simulink model "ElectricalCoupling_testing"  (R2024b)
settings: Solver=FixedStepAuto  StartTime=0.0  StopTime=20  RelTol=1e-3
undefined symbols (not defined in the file): ac4b, c4e6, DiscIntNeverNeededParam
libraries: fl_lib x22, nesl_utility x21, ee_lib x5, simulink x3
(part 2 of 2)

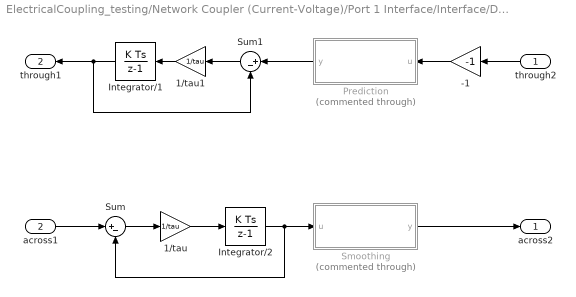
== system ElectricalCoupling_testing/Network Coupler (Current-Voltage)/Port 1 Interface/Interface/Discrete ==
  through2 : Inport
  across1 : Inport  Port=2
  -1 : Gain  Gain=-1  SaturateOnIntegerOverflow=on  OutDataTypeStr=Inherit: Same as input  ParamDataTypeStr=Inherit: Same as input
  1/tau : Gain  Gain=1/tau  SaturateOnIntegerOverflow=on  OutDataTypeStr=Inherit: Same as input  ParamDataTypeStr=Inherit: Same as input
  1/tau1 : Gain  Gain=1/tau  SaturateOnIntegerOverflow=on  OutDataTypeStr=Inherit: Same as input  ParamDataTypeStr=Inherit: Same as input
  Integrator/1 : DiscreteIntegrator  InitialCondition=i0  SampleTime=h1  ICPrevOutput=DiscIntNeverNeededParam  ICPrevScaledInput=DiscIntNeverNeededParam
  Integrator/2 : DiscreteIntegrator  InitialCondition=v0  SampleTime=h1  ICPrevOutput=DiscIntNeverNeededParam  ICPrevScaledInput=DiscIntNeverNeededParam
  Prediction : Subsystem  Commented=through  mask(Prediction (slow->fast)){h2=h2, h1=h1}
      mask prompts: h2 "physmod:simscape:couplers:SimscapeNetworkCouplersLib:PortUDiscreteSampleTimes_MP"; h1 "physmod:simscape:couplers:SimscapeNetworkCouplersLib:PortYDiscreteSampleTimes_MP"
      mask help: physmod:simscape:couplers:SimscapeNetworkCouplersLib:Predictionslowfast_MD
      mask DialogControl h2 Prompt: Port u discrete sample time (s)
      mask DialogControl h1 Prompt: Port y discrete sample time (s)
  Smoothing : Subsystem  Commented=through  mask(Smoothing (fast->slow)){nSmooth=nSmooth, h1=h1, smoothing0=v0}
      mask prompts: nSmooth "physmod:simscape:couplers:SimscapeNetworkCouplersLib:NumberOfSamplesOverWhichToSmooth_MP"; h1 "physmod:simscape:couplers:SimscapeNetworkCouplersLib:PortUDiscreteSampleTimes_MP"; smoothing0 "physmod:simscape:couplers:SimscapeNetworkCouplersLib:InitialOutput_MP"
      mask help: physmod:simscape:couplers:SimscapeNetworkCouplersLib:Smoothingfastslow_MD
      mask DialogControl nSmooth Prompt: Number of samples over which to smooth
      mask DialogControl h1 Prompt: Port u discrete sample time (s)
      mask DialogControl smoothing0 Prompt: Initial output
  Sum : Sum  Inputs=|+-  InputSameDT=on  SaturateOnIntegerOverflow=on  OutDataTypeStr=Inherit: Same as first input
  Sum1 : Sum  Inputs=|+-  InputSameDT=on  SaturateOnIntegerOverflow=on  OutDataTypeStr=Inherit: Same as first input
  across2 : Outport
  through1 : Outport  Port=2
  wires:
  Smoothing/1(y) -> across2/1
  -1/1 -> Prediction/1(u)
  through2/1 -> -1/1
  Prediction/1(y) -> Sum1/1
  Sum1/1 -> 1/tau1/1
  Integrator/1/1 -> through1/1, Sum1/2
  Integrator/2/1 -> Sum/2, Smoothing/1(u)
  Sum/1 -> 1/tau/1
  1/tau1/1 -> Integrator/1/1
  1/tau/1 -> Integrator/2/1
  across1/1 -> Sum/1

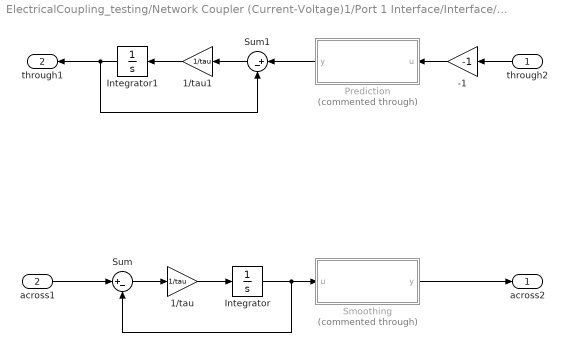
== system ElectricalCoupling_testing/Network Coupler (Current-Voltage)1/Port 1 Interface/Interface/Continuous ==
  through2 : Inport
  across1 : Inport  Port=2
  -1 : Gain  Gain=-1  SaturateOnIntegerOverflow=on  OutDataTypeStr=Inherit: Same as input  ParamDataTypeStr=Inherit: Same as input
  1/tau : Gain  Gain=1/tau  SaturateOnIntegerOverflow=on  OutDataTypeStr=Inherit: Same as input  ParamDataTypeStr=Inherit: Same as input
  1/tau1 : Gain  Gain=1/tau  SaturateOnIntegerOverflow=on  OutDataTypeStr=Inherit: Same as input  ParamDataTypeStr=Inherit: Same as input
  Integrator : Integrator  InitialCondition=v0
  Integrator1 : Integrator  InitialCondition=i0
  Prediction : Subsystem  Commented=through  mask(Prediction (discrete->continuous)){h2=h2}
      mask prompts: h2 "physmod:simscape:couplers:SimscapeNetworkCouplersLib:PortUDiscreteSampleTimes_MP"
      mask help: physmod:simscape:couplers:SimscapeNetworkCouplersLib:Predictiondiscretecontinuous_MD
      mask DialogControl h2 Prompt: Port u discrete sample time (s)
  Smoothing : Subsystem  Commented=through  mask(Smoothing (continuous->discrete)){tsSmoothing=tsSmoothing, smoothing0=v0}
      mask prompts: tsSmoothing "physmod:simscape:couplers:SimscapeNetworkCouplersLib:SmoothingTimeConstants_MP"; smoothing0 "physmod:simscape:couplers:SimscapeNetworkCouplersLib:InitialOutput_MP"
      mask help: physmod:simscape:couplers:SimscapeNetworkCouplersLib:Smoothingcontinuousdiscrete_MD
      mask DialogControl tsSmoothing Prompt: Smoothing time constant (s)
      mask DialogControl smoothing0 Prompt: Initial output
  Sum : Sum  Inputs=|+-  InputSameDT=on  SaturateOnIntegerOverflow=on  OutDataTypeStr=Inherit: Same as first input
  Sum1 : Sum  Inputs=|+-  InputSameDT=on  SaturateOnIntegerOverflow=on  OutDataTypeStr=Inherit: Same as first input
  across2 : Outport
  through1 : Outport  Port=2
  wires:
  Prediction/1(y) -> Sum1/1
  Sum1/1 -> 1/tau1/1
  1/tau1/1 -> Integrator1/1
  Integrator1/1 -> through1/1, Sum1/2
  across1/1 -> Sum/1
  Integrator/1 -> Smoothing/1(u), Sum/2
  Sum/1 -> 1/tau/1
  1/tau/1 -> Integrator/1
  through2/1 -> -1/1
  -1/1 -> Prediction/1(u)
  Smoothing/1(y) -> across2/1

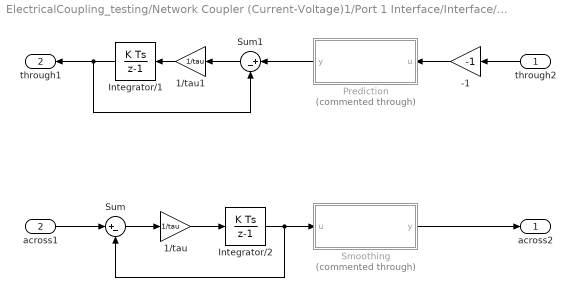
== system ElectricalCoupling_testing/Network Coupler (Current-Voltage)1/Port 1 Interface/Interface/Discrete ==
  through2 : Inport
  across1 : Inport  Port=2
  -1 : Gain  Gain=-1  SaturateOnIntegerOverflow=on  OutDataTypeStr=Inherit: Same as input  ParamDataTypeStr=Inherit: Same as input
  1/tau : Gain  Gain=1/tau  SaturateOnIntegerOverflow=on  OutDataTypeStr=Inherit: Same as input  ParamDataTypeStr=Inherit: Same as input
  1/tau1 : Gain  Gain=1/tau  SaturateOnIntegerOverflow=on  OutDataTypeStr=Inherit: Same as input  ParamDataTypeStr=Inherit: Same as input
  Integrator/1 : DiscreteIntegrator  InitialCondition=i0  SampleTime=h1  ICPrevOutput=DiscIntNeverNeededParam  ICPrevScaledInput=DiscIntNeverNeededParam
  Integrator/2 : DiscreteIntegrator  InitialCondition=v0  SampleTime=h1  ICPrevOutput=DiscIntNeverNeededParam  ICPrevScaledInput=DiscIntNeverNeededParam
  Prediction : Subsystem  Commented=through  mask(Prediction (slow->fast)){h2=h2, h1=h1}
      mask prompts: h2 "physmod:simscape:couplers:SimscapeNetworkCouplersLib:PortUDiscreteSampleTimes_MP"; h1 "physmod:simscape:couplers:SimscapeNetworkCouplersLib:PortYDiscreteSampleTimes_MP"
      mask help: physmod:simscape:couplers:SimscapeNetworkCouplersLib:Predictionslowfast_MD
      mask DialogControl h2 Prompt: Port u discrete sample time (s)
      mask DialogControl h1 Prompt: Port y discrete sample time (s)
  Smoothing : Subsystem  Commented=through  mask(Smoothing (fast->slow)){nSmooth=nSmooth, h1=h1, smoothing0=v0}
      mask prompts: nSmooth "physmod:simscape:couplers:SimscapeNetworkCouplersLib:NumberOfSamplesOverWhichToSmooth_MP"; h1 "physmod:simscape:couplers:SimscapeNetworkCouplersLib:PortUDiscreteSampleTimes_MP"; smoothing0 "physmod:simscape:couplers:SimscapeNetworkCouplersLib:InitialOutput_MP"
      mask help: physmod:simscape:couplers:SimscapeNetworkCouplersLib:Smoothingfastslow_MD
      mask DialogControl nSmooth Prompt: Number of samples over which to smooth
      mask DialogControl h1 Prompt: Port u discrete sample time (s)
      mask DialogControl smoothing0 Prompt: Initial output
  Sum : Sum  Inputs=|+-  InputSameDT=on  SaturateOnIntegerOverflow=on  OutDataTypeStr=Inherit: Same as first input
  Sum1 : Sum  Inputs=|+-  InputSameDT=on  SaturateOnIntegerOverflow=on  OutDataTypeStr=Inherit: Same as first input
  across2 : Outport
  through1 : Outport  Port=2
  wires:
  across1/1 -> Sum/1
  1/tau/1 -> Integrator/2/1
  1/tau1/1 -> Integrator/1/1
  Sum/1 -> 1/tau/1
  Integrator/2/1 -> Smoothing/1(u), Sum/2
  Integrator/1/1 -> Sum1/2, through1/1
  Sum1/1 -> 1/tau1/1
  Prediction/1(y) -> Sum1/1
  through2/1 -> -1/1
  -1/1 -> Prediction/1(u)
  Smoothing/1(y) -> across2/1

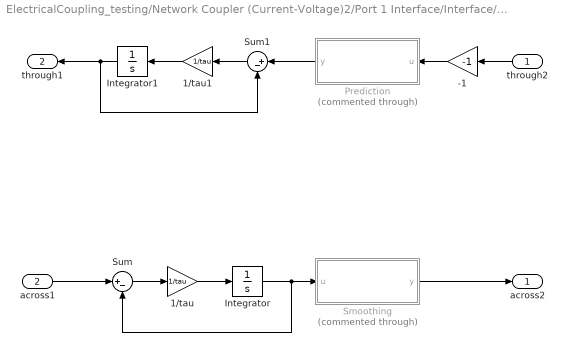
== system ElectricalCoupling_testing/Network Coupler (Current-Voltage)2/Port 1 Interface/Interface/Continuous ==
  through2 : Inport
  across1 : Inport  Port=2
  -1 : Gain  Gain=-1  SaturateOnIntegerOverflow=on  OutDataTypeStr=Inherit: Same as input  ParamDataTypeStr=Inherit: Same as input
  1/tau : Gain  Gain=1/tau  SaturateOnIntegerOverflow=on  OutDataTypeStr=Inherit: Same as input  ParamDataTypeStr=Inherit: Same as input
  1/tau1 : Gain  Gain=1/tau  SaturateOnIntegerOverflow=on  OutDataTypeStr=Inherit: Same as input  ParamDataTypeStr=Inherit: Same as input
  Integrator : Integrator  InitialCondition=v0
  Integrator1 : Integrator  InitialCondition=i0
  Prediction : Subsystem  Commented=through  mask(Prediction (discrete->continuous)){h2=h2}
      mask prompts: h2 "physmod:simscape:couplers:SimscapeNetworkCouplersLib:PortUDiscreteSampleTimes_MP"
      mask help: physmod:simscape:couplers:SimscapeNetworkCouplersLib:Predictiondiscretecontinuous_MD
      mask DialogControl h2 Prompt: Port u discrete sample time (s)
  Smoothing : Subsystem  Commented=through  mask(Smoothing (continuous->discrete)){tsSmoothing=tsSmoothing, smoothing0=v0}
      mask prompts: tsSmoothing "physmod:simscape:couplers:SimscapeNetworkCouplersLib:SmoothingTimeConstants_MP"; smoothing0 "physmod:simscape:couplers:SimscapeNetworkCouplersLib:InitialOutput_MP"
      mask help: physmod:simscape:couplers:SimscapeNetworkCouplersLib:Smoothingcontinuousdiscrete_MD
      mask DialogControl tsSmoothing Prompt: Smoothing time constant (s)
      mask DialogControl smoothing0 Prompt: Initial output
  Sum : Sum  Inputs=|+-  InputSameDT=on  SaturateOnIntegerOverflow=on  OutDataTypeStr=Inherit: Same as first input
  Sum1 : Sum  Inputs=|+-  InputSameDT=on  SaturateOnIntegerOverflow=on  OutDataTypeStr=Inherit: Same as first input
  across2 : Outport
  through1 : Outport  Port=2
  wires:
  Smoothing/1(y) -> across2/1
  -1/1 -> Prediction/1(u)
  through2/1 -> -1/1
  1/tau/1 -> Integrator/1
  Sum/1 -> 1/tau/1
  Integrator/1 -> Sum/2, Smoothing/1(u)
  across1/1 -> Sum/1
  Integrator1/1 -> Sum1/2, through1/1
  1/tau1/1 -> Integrator1/1
  Sum1/1 -> 1/tau1/1
  Prediction/1(y) -> Sum1/1

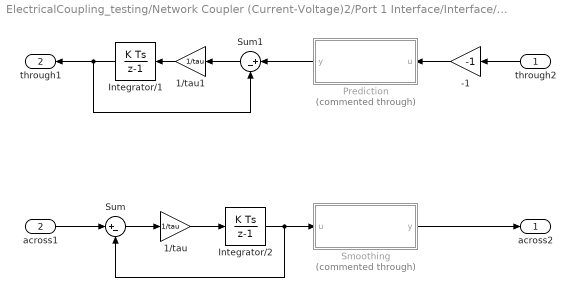
== system ElectricalCoupling_testing/Network Coupler (Current-Voltage)2/Port 1 Interface/Interface/Discrete ==
  through2 : Inport
  across1 : Inport  Port=2
  -1 : Gain  Gain=-1  SaturateOnIntegerOverflow=on  OutDataTypeStr=Inherit: Same as input  ParamDataTypeStr=Inherit: Same as input
  1/tau : Gain  Gain=1/tau  SaturateOnIntegerOverflow=on  OutDataTypeStr=Inherit: Same as input  ParamDataTypeStr=Inherit: Same as input
  1/tau1 : Gain  Gain=1/tau  SaturateOnIntegerOverflow=on  OutDataTypeStr=Inherit: Same as input  ParamDataTypeStr=Inherit: Same as input
  Integrator/1 : DiscreteIntegrator  InitialCondition=i0  SampleTime=h1  ICPrevOutput=DiscIntNeverNeededParam  ICPrevScaledInput=DiscIntNeverNeededParam
  Integrator/2 : DiscreteIntegrator  InitialCondition=v0  SampleTime=h1  ICPrevOutput=DiscIntNeverNeededParam  ICPrevScaledInput=DiscIntNeverNeededParam
  Prediction : Subsystem  Commented=through  mask(Prediction (slow->fast)){h2=h2, h1=h1}
      mask prompts: h2 "physmod:simscape:couplers:SimscapeNetworkCouplersLib:PortUDiscreteSampleTimes_MP"; h1 "physmod:simscape:couplers:SimscapeNetworkCouplersLib:PortYDiscreteSampleTimes_MP"
      mask help: physmod:simscape:couplers:SimscapeNetworkCouplersLib:Predictionslowfast_MD
      mask DialogControl h2 Prompt: Port u discrete sample time (s)
      mask DialogControl h1 Prompt: Port y discrete sample time (s)
  Smoothing : Subsystem  Commented=through  mask(Smoothing (fast->slow)){nSmooth=nSmooth, h1=h1, smoothing0=v0}
      mask prompts: nSmooth "physmod:simscape:couplers:SimscapeNetworkCouplersLib:NumberOfSamplesOverWhichToSmooth_MP"; h1 "physmod:simscape:couplers:SimscapeNetworkCouplersLib:PortUDiscreteSampleTimes_MP"; smoothing0 "physmod:simscape:couplers:SimscapeNetworkCouplersLib:InitialOutput_MP"
      mask help: physmod:simscape:couplers:SimscapeNetworkCouplersLib:Smoothingfastslow_MD
      mask DialogControl nSmooth Prompt: Number of samples over which to smooth
      mask DialogControl h1 Prompt: Port u discrete sample time (s)
      mask DialogControl smoothing0 Prompt: Initial output
  Sum : Sum  Inputs=|+-  InputSameDT=on  SaturateOnIntegerOverflow=on  OutDataTypeStr=Inherit: Same as first input
  Sum1 : Sum  Inputs=|+-  InputSameDT=on  SaturateOnIntegerOverflow=on  OutDataTypeStr=Inherit: Same as first input
  across2 : Outport
  through1 : Outport  Port=2
  wires:
  Smoothing/1(y) -> across2/1
  -1/1 -> Prediction/1(u)
  through2/1 -> -1/1
  Prediction/1(y) -> Sum1/1
  Sum1/1 -> 1/tau1/1
  Integrator/1/1 -> through1/1, Sum1/2
  Integrator/2/1 -> Sum/2, Smoothing/1(u)
  Sum/1 -> 1/tau/1
  1/tau1/1 -> Integrator/1/1
  1/tau/1 -> Integrator/2/1
  across1/1 -> Sum/1

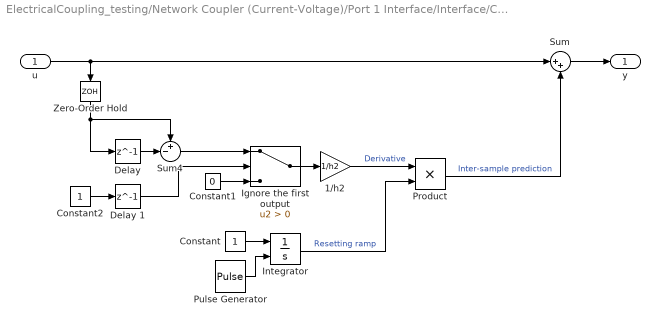
== system ElectricalCoupling_testing/Network Coupler (Current-Voltage)/Port 1 Interface/Interface/Continuous/Prediction ==
  u : Inport
  1/h2 : Gain  Gain=1/h2
  Constant : Constant  SampleTime=h2
  Constant1 : Constant  Value=0  SampleTime=h2
  Constant2 : Constant  SampleTime=h2
  "Delay " : Delay  DelayLength=1  SampleTime=h2
  Delay 1 : Delay  DelayLength=1  SampleTime=h2
  Ignore the first output : Switch  Criteria=u2 > Threshold  SaturateOnIntegerOverflow=off  InputSameDT=off
  Integrator : Integrator  ExternalReset=either  LimitOutput=on  UpperSaturationLimit=1  LowerSaturationLimit=0
  Product : Product
  Pulse Generator : DiscretePulseGenerator  SampleTime=h2
  Sum : Sum  Inputs=|++
  Sum4 : Sum  Inputs=+-|
  Zero-Order Hold : ZeroOrderHold  SampleTime=h2
  y : Outport
  wires:
  Constant2/1 -> Delay 1/1
  Delay 1/1 -> Ignore the first output/2
  Constant1/1 -> Ignore the first output/3
  Sum4/1 -> Ignore the first output/1
  Ignore the first output/1 -> 1/h2/1
  Pulse Generator/1 -> Integrator/2
  Constant/1 -> Integrator/1
  Integrator/1 -> Product/2  "Resetting ramp"
  Sum/1 -> y/1
  1/h2/1 -> Product/1  "Derivative"
  "Delay "/1 -> Sum4/2
  u/1 -> Zero-Order Hold/1, Sum/1
  Zero-Order Hold/1 -> "Delay "/1, Sum4/1
  Product/1 -> Sum/2  "Inter-sample prediction"

== system ElectricalCoupling_testing/Network Coupler (Current-Voltage)/Port 1 Interface/Interface/Continuous/Smoothing ==
  u : Inport
  Gain : Gain  Gain=1/tsSmoothing
  Integrator : Integrator  InitialCondition=smoothing0
  Sum : Sum  Inputs=|+-
  y : Outport
  wires:
  Sum/1 -> Gain/1
  Gain/1 -> Integrator/1
  Integrator/1 -> y/1, Sum/2
  u/1 -> Sum/1

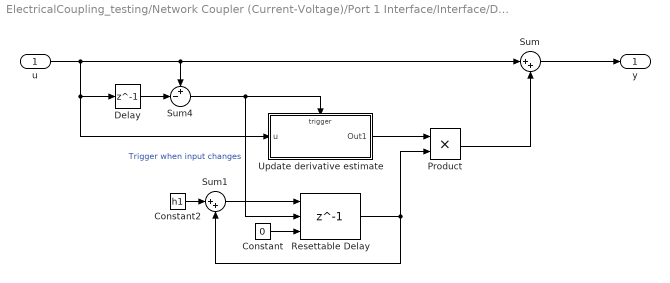
== system ElectricalCoupling_testing/Network Coupler (Current-Voltage)/Port 1 Interface/Interface/Discrete/Prediction ==
  u : Inport
  Constant : Constant  Value=0  SampleTime=h1
  Constant2 : Constant  Value=h1  SampleTime=h1
  "Delay " : Delay  DelayLength=1  SampleTime=h1
  Product : Product
  Resettable Delay : Delay  DelayLength=1  InitialConditionSource=Input port  ExternalReset=Rising  SampleTime=h1
      settings: InputPortMap=u0,r5,p4
  Sum : Sum  Inputs=|++
  Sum1 : Sum  Inputs=|++
  Sum4 : Sum  Inputs=+-|
  Update derivative estimate : Subsystem  TreatAsAtomicUnit=on
  y : Outport
  wires:
  Update derivative estimate/1(Out1) -> Product/1
  u/1 -> Sum/1, Sum4/1, Update derivative estimate/1(u), "Delay "/1
  "Delay "/1 -> Sum4/2
  Sum4/1 -> Update derivative estimate/Trigger, Resettable Delay/2  "Trigger when input changes"
  Sum1/1 -> Resettable Delay/1
  Resettable Delay/1 -> Product/2, Sum1/2
  Constant2/1 -> Sum1/1
  Constant/1 -> Resettable Delay/3
  Sum/1 -> y/1
  Product/1 -> Sum/2

== system ElectricalCoupling_testing/Network Coupler (Current-Voltage)/Port 1 Interface/Interface/Discrete/Smoothing ==
  u : Inport
  Gain : Gain  Gain=1/nSmooth
  Sum of Elements : Sum  Inputs=+
  Tapped Delay : simulink/Discrete/Tapped Delay  vinit=smoothing0  samptime=h1  NumDelays=nSmooth  DelayOrder=Oldest  includeCurrent=off
  y : Outport
  wires:
  u/1 -> Tapped Delay/1
  Tapped Delay/1 -> Sum of Elements/1
  Sum of Elements/1 -> Gain/1
  Gain/1 -> y/1

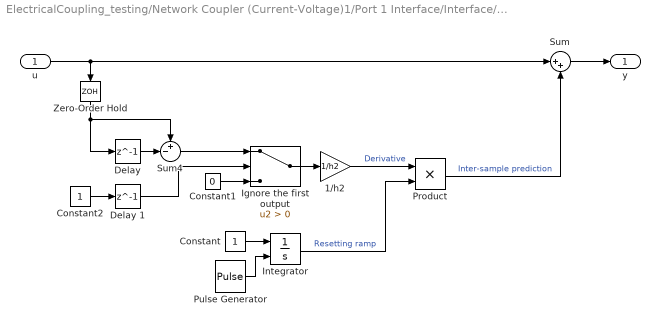
== system ElectricalCoupling_testing/Network Coupler (Current-Voltage)1/Port 1 Interface/Interface/Continuous/Prediction ==
  u : Inport
  1/h2 : Gain  Gain=1/h2
  Constant : Constant  SampleTime=h2
  Constant1 : Constant  Value=0  SampleTime=h2
  Constant2 : Constant  SampleTime=h2
  "Delay " : Delay  DelayLength=1  SampleTime=h2
  Delay 1 : Delay  DelayLength=1  SampleTime=h2
  Ignore the first output : Switch  Criteria=u2 > Threshold  SaturateOnIntegerOverflow=off  InputSameDT=off
  Integrator : Integrator  ExternalReset=either  LimitOutput=on  UpperSaturationLimit=1  LowerSaturationLimit=0
  Product : Product
  Pulse Generator : DiscretePulseGenerator  SampleTime=h2
  Sum : Sum  Inputs=|++
  Sum4 : Sum  Inputs=+-|
  Zero-Order Hold : ZeroOrderHold  SampleTime=h2
  y : Outport
  wires:
  Product/1 -> Sum/2  "Inter-sample prediction"
  Zero-Order Hold/1 -> Sum4/1, "Delay "/1
  u/1 -> Sum/1, Zero-Order Hold/1
  "Delay "/1 -> Sum4/2
  1/h2/1 -> Product/1  "Derivative"
  Sum/1 -> y/1
  Integrator/1 -> Product/2  "Resetting ramp"
  Constant/1 -> Integrator/1
  Pulse Generator/1 -> Integrator/2
  Ignore the first output/1 -> 1/h2/1
  Sum4/1 -> Ignore the first output/1
  Constant1/1 -> Ignore the first output/3
  Delay 1/1 -> Ignore the first output/2
  Constant2/1 -> Delay 1/1

== system ElectricalCoupling_testing/Network Coupler (Current-Voltage)1/Port 1 Interface/Interface/Continuous/Smoothing ==
  u : Inport
  Gain : Gain  Gain=1/tsSmoothing
  Integrator : Integrator  InitialCondition=smoothing0
  Sum : Sum  Inputs=|+-
  y : Outport
  wires:
  u/1 -> Sum/1
  Integrator/1 -> Sum/2, y/1
  Gain/1 -> Integrator/1
  Sum/1 -> Gain/1

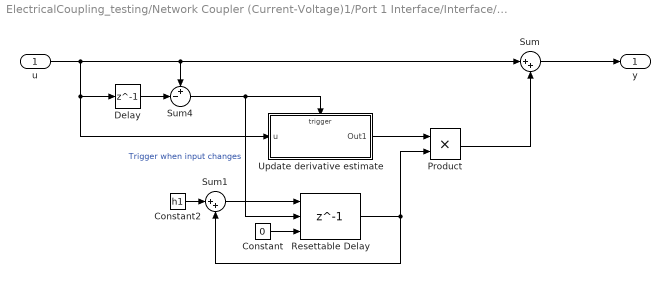
== system ElectricalCoupling_testing/Network Coupler (Current-Voltage)1/Port 1 Interface/Interface/Discrete/Prediction ==
  u : Inport
  Constant : Constant  Value=0  SampleTime=h1
  Constant2 : Constant  Value=h1  SampleTime=h1
  "Delay " : Delay  DelayLength=1  SampleTime=h1
  Product : Product
  Resettable Delay : Delay  DelayLength=1  InitialConditionSource=Input port  ExternalReset=Rising  SampleTime=h1
      settings: InputPortMap=u0,r5,p4
  Sum : Sum  Inputs=|++
  Sum1 : Sum  Inputs=|++
  Sum4 : Sum  Inputs=+-|
  Update derivative estimate : Subsystem  TreatAsAtomicUnit=on
  y : Outport
  wires:
  Product/1 -> Sum/2
  Sum/1 -> y/1
  Constant/1 -> Resettable Delay/3
  Constant2/1 -> Sum1/1
  Resettable Delay/1 -> Sum1/2, Product/2
  Sum1/1 -> Resettable Delay/1
  Sum4/1 -> Resettable Delay/2, Update derivative estimate/Trigger  "Trigger when input changes"
  "Delay "/1 -> Sum4/2
  u/1 -> "Delay "/1, Update derivative estimate/1(u), Sum4/1, Sum/1
  Update derivative estimate/1(Out1) -> Product/1

== system ElectricalCoupling_testing/Network Coupler (Current-Voltage)1/Port 1 Interface/Interface/Discrete/Smoothing ==
  u : Inport
  Gain : Gain  Gain=1/nSmooth
  Sum of Elements : Sum  Inputs=+
  Tapped Delay : simulink/Discrete/Tapped Delay  vinit=smoothing0  samptime=h1  NumDelays=nSmooth  DelayOrder=Oldest  includeCurrent=off
  y : Outport
  wires:
  Gain/1 -> y/1
  Sum of Elements/1 -> Gain/1
  Tapped Delay/1 -> Sum of Elements/1
  u/1 -> Tapped Delay/1

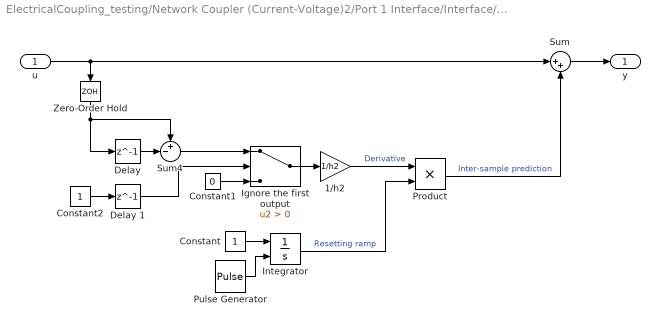
== system ElectricalCoupling_testing/Network Coupler (Current-Voltage)2/Port 1 Interface/Interface/Continuous/Prediction ==
  u : Inport
  1/h2 : Gain  Gain=1/h2
  Constant : Constant  SampleTime=h2
  Constant1 : Constant  Value=0  SampleTime=h2
  Constant2 : Constant  SampleTime=h2
  "Delay " : Delay  DelayLength=1  SampleTime=h2
  Delay 1 : Delay  DelayLength=1  SampleTime=h2
  Ignore the first output : Switch  Criteria=u2 > Threshold  SaturateOnIntegerOverflow=off  InputSameDT=off
  Integrator : Integrator  ExternalReset=either  LimitOutput=on  UpperSaturationLimit=1  LowerSaturationLimit=0
  Product : Product
  Pulse Generator : DiscretePulseGenerator  SampleTime=h2
  Sum : Sum  Inputs=|++
  Sum4 : Sum  Inputs=+-|
  Zero-Order Hold : ZeroOrderHold  SampleTime=h2
  y : Outport
  wires:
  Constant2/1 -> Delay 1/1
  Delay 1/1 -> Ignore the first output/2
  Constant1/1 -> Ignore the first output/3
  Sum4/1 -> Ignore the first output/1
  Ignore the first output/1 -> 1/h2/1
  Pulse Generator/1 -> Integrator/2
  Constant/1 -> Integrator/1
  Integrator/1 -> Product/2  "Resetting ramp"
  Sum/1 -> y/1
  1/h2/1 -> Product/1  "Derivative"
  "Delay "/1 -> Sum4/2
  u/1 -> Zero-Order Hold/1, Sum/1
  Zero-Order Hold/1 -> "Delay "/1, Sum4/1
  Product/1 -> Sum/2  "Inter-sample prediction"

== system ElectricalCoupling_testing/Network Coupler (Current-Voltage)2/Port 1 Interface/Interface/Continuous/Smoothing ==
  u : Inport
  Gain : Gain  Gain=1/tsSmoothing
  Integrator : Integrator  InitialCondition=smoothing0
  Sum : Sum  Inputs=|+-
  y : Outport
  wires:
  Sum/1 -> Gain/1
  Gain/1 -> Integrator/1
  Integrator/1 -> y/1, Sum/2
  u/1 -> Sum/1

== system ElectricalCoupling_testing/Network Coupler (Current-Voltage)2/Port 1 Interface/Interface/Discrete/Prediction ==
  u : Inport
  Constant : Constant  Value=0  SampleTime=h1
  Constant2 : Constant  Value=h1  SampleTime=h1
  "Delay " : Delay  DelayLength=1  SampleTime=h1
  Product : Product
  Resettable Delay : Delay  DelayLength=1  InitialConditionSource=Input port  ExternalReset=Rising  SampleTime=h1
      settings: InputPortMap=u0,r5,p4
  Sum : Sum  Inputs=|++
  Sum1 : Sum  Inputs=|++
  Sum4 : Sum  Inputs=+-|
  Update derivative estimate : Subsystem  TreatAsAtomicUnit=on
  y : Outport
  wires:
  Update derivative estimate/1(Out1) -> Product/1
  u/1 -> Sum/1, Sum4/1, Update derivative estimate/1(u), "Delay "/1
  "Delay "/1 -> Sum4/2
  Sum4/1 -> Update derivative estimate/Trigger, Resettable Delay/2  "Trigger when input changes"
  Sum1/1 -> Resettable Delay/1
  Resettable Delay/1 -> Product/2, Sum1/2
  Constant2/1 -> Sum1/1
  Constant/1 -> Resettable Delay/3
  Sum/1 -> y/1
  Product/1 -> Sum/2

== system ElectricalCoupling_testing/Network Coupler (Current-Voltage)2/Port 1 Interface/Interface/Discrete/Smoothing ==
  u : Inport
  Gain : Gain  Gain=1/nSmooth
  Sum of Elements : Sum  Inputs=+
  Tapped Delay : simulink/Discrete/Tapped Delay  vinit=smoothing0  samptime=h1  NumDelays=nSmooth  DelayOrder=Oldest  includeCurrent=off
  y : Outport
  wires:
  u/1 -> Tapped Delay/1
  Tapped Delay/1 -> Sum of Elements/1
  Sum of Elements/1 -> Gain/1
  Gain/1 -> y/1

== system ElectricalCoupling_testing/Network Coupler (Current-Voltage)/Port 1 Interface/Interface/Discrete/Prediction/Update derivative estimate ==
  u : Inport
  Trigger : TriggerPort  VariantControl=(inherit)
  1/h2 : Gain  Gain=1/h2
  Constant : Constant  Value=0  SampleTime=-1
  Constant1 : Constant  SampleTime=-1
  Sum : Sum  Inputs=|-+
  Switch : Switch  Criteria=u2 > Threshold  SaturateOnIntegerOverflow=off  InputSameDT=off
  Unit Delay : UnitDelay  SampleTime=-1  HasFrameUpgradeWarning=on
  Wait one sample : UnitDelay  SampleTime=-1  HasFrameUpgradeWarning=on
  Out1 : Outport
  wires:
  Constant1/1 -> Wait one sample/1
  Wait one sample/1 -> Switch/2
  Constant/1 -> Switch/3
  Sum/1 -> Switch/1
  Switch/1 -> 1/h2/1
  1/h2/1 -> Out1/1
  u/1 -> Sum/2, Unit Delay/1
  Unit Delay/1 -> Sum/1

== system ElectricalCoupling_testing/Network Coupler (Current-Voltage)1/Port 1 Interface/Interface/Discrete/Prediction/Update derivative estimate ==
  u : Inport
  Trigger : TriggerPort  VariantControl=(inherit)
  1/h2 : Gain  Gain=1/h2
  Constant : Constant  Value=0  SampleTime=-1
  Constant1 : Constant  SampleTime=-1
  Sum : Sum  Inputs=|-+
  Switch : Switch  Criteria=u2 > Threshold  SaturateOnIntegerOverflow=off  InputSameDT=off
  Unit Delay : UnitDelay  SampleTime=-1  HasFrameUpgradeWarning=on
  Wait one sample : UnitDelay  SampleTime=-1  HasFrameUpgradeWarning=on
  Out1 : Outport
  wires:
  Unit Delay/1 -> Sum/1
  u/1 -> Unit Delay/1, Sum/2
  1/h2/1 -> Out1/1
  Switch/1 -> 1/h2/1
  Sum/1 -> Switch/1
  Constant/1 -> Switch/3
  Wait one sample/1 -> Switch/2
  Constant1/1 -> Wait one sample/1

== system ElectricalCoupling_testing/Network Coupler (Current-Voltage)2/Port 1 Interface/Interface/Discrete/Prediction/Update derivative estimate ==
  u : Inport
  Trigger : TriggerPort  VariantControl=(inherit)
  1/h2 : Gain  Gain=1/h2
  Constant : Constant  Value=0  SampleTime=-1
  Constant1 : Constant  SampleTime=-1
  Sum : Sum  Inputs=|-+
  Switch : Switch  Criteria=u2 > Threshold  SaturateOnIntegerOverflow=off  InputSameDT=off
  Unit Delay : UnitDelay  SampleTime=-1  HasFrameUpgradeWarning=on
  Wait one sample : UnitDelay  SampleTime=-1  HasFrameUpgradeWarning=on
  Out1 : Outport
  wires:
  Constant1/1 -> Wait one sample/1
  Wait one sample/1 -> Switch/2
  Constant/1 -> Switch/3
  Sum/1 -> Switch/1
  Switch/1 -> 1/h2/1
  1/h2/1 -> Out1/1
  u/1 -> Sum/2, Unit Delay/1
  Unit Delay/1 -> Sum/1
